simulink model "VSDk_PMSM_6"  (R2024a)
settings: Solver=VariableStepAuto  StartTime=0.0  StopTime=10.0  RelTol=1e-3
values from neighbouring files (symbols this model uses):
  faif = 0.1351    [init.m]
  Iq_limit = Tn/(1.5*p*faif)*1    (= 90.6192943499)    [init.m]
  Jm = 0.36    [init.m]
  Ki_id_vsd = Rs * wc    (= 61.7197292724)    [init.m]
  Ki_iq_vsd = Rs * wc    (= 61.7197292724)    [init.m]
  Ki_x = Rs * wc_xy    (= 61.7197292724)    [init.m]
  Ki_y = Rs * wc_xy    (= 61.7197292724)    [init.m]
  Kis_vsd = (ws^2 * Jm) / KT    (= 438.324399752)    [init.m]
  Kp_id_vsd = Ld_eff * wc    (= 0.485061905714)    [init.m]
  Kp_iq_vsd = Lq_eff * wc    (= 0.485061905714)    [init.m]
  Kp_x = Lx * wc_xy    (= 0.020106192983)    [init.m]
  Kp_y = Ly * wc_xy    (= 0.020106192983)    [init.m]
  Kps_vsd = (2 * zeta * ws * Jm) / KT    (= 19.7285507573)    [init.m]
  LD = Ld+Ldd    (= 7.72e-05)    [init.m]
  Ld = 40.2e-6    (= 4.02e-05)    [init.m]
  Ldd = 37e-6    (= 3.7e-05)    [init.m]
  Ldz = Ld-Ldd    (= 3.2e-06)    [init.m]
  LQ = Lq+Lqq    (= 7.72e-05)    [init.m]
  Lq = 40.2e-6    (= 4.02e-05)    [init.m]
  Lqq = 37e-6    (= 3.7e-05)    [init.m]
  n = 2000    [init.m]
  p = 4    [init.m]
  Rs = 9.823e-3    (= 0.009823)    [init.m]
  Tn = 734.56/10    (= 73.456)    [init.m]
  Ts = 1/(16e3)    (= 6.25e-05)    [init.m]
  Ts_FEA = 1e-7    (= 1e-07)    [init.m]
  VDC = 1200    [init.m]
  wc_xy = 2 * pi * fc_xy    (= 6283.18530718)    [init.m]
libraries: spsIGBTDiodeLib x24, spsVoltageMeasurementLib x16, spsSeriesRLCBranchLib x12, spsDiodeLib x12, spsOnDelayLib x12, slpidlib x11, simulink x7, spsControlledCurrentSourceLib x6, spsDCVoltageSourceLib x1, spsdq0toAlphaBetaZeroLib x1, spspowerguiLib x1
(part 3 of 3)

== matlab function VSDk_PMSM_6/Subsystem2/NTSV_9_nearest2 ==
  data: Alpha input; Beta input; Ta1 output; Ta2 output; Tb1 output; Tb2 output; Tc1 output; Tc2 output; r input; VecSector1 output
function [Ta1,Ta2,Tb1,Tb2,Tc1,Tc2,VecSector1]  = fcn(Alpha,Beta,r)
temp1=Beta;
temp2=0.8660254*Alpha+Beta*0.5;
temp3=temp2-temp1;
%0.8660254*Alpha-0.5beta
%temp1+temp2 0.8660254*Alpha+1.5beta
%temp3+temp2 2*0.8660254*Alpha
%temp1-temp3 -0.8660254*Alpha+1.5beta
VecSector1=3;
VecSector2=1;
VecSector3=0;


if temp2>0
    VecSector1=VecSector1-1;
end
if temp3>0
    VecSector1=VecSector1-1;
end
if temp1<0
    VecSector1=7-VecSector1;
end 


switch VecSector1
    case {1,4}  
       if(abs(temp2)>0.5)
           VecSector2=VecSector2+1;
           if(abs(temp3)<0.5)
               VecSector2=VecSector2+1;
               if(abs(temp1)>0.5)
                   VecSector2=VecSector2+1;
               end
           end
       end
       if(temp1<temp3)
           VecSector3=1;
       else
           VecSector3=2;
       end
    case {2,5}
       if(abs(temp1)>0.5)
           VecSector2=VecSector2+1;
           if(abs(temp2)<0.5)
               VecSector2=VecSector2+1;
               if(abs(temp3)>0.5)
                   VecSector2=VecSector2+1;
               end
           end
       end
       if(temp2+temp3>0)
          VecSector3=1;
       else
           VecSector3=2;
       end 
    case {3,6}
       if(abs(temp3)>0.5)
           VecSector2=VecSector2+1;
           if(abs(temp1)<0.5)
               VecSector2=VecSector2+1;
               if(abs(temp2)>0.5)
                   VecSector2=VecSector2+1;
               end
           end
       end
       if(temp1+temp2>0)
          VecSector3=1;
       else
           VecSector3=2;
       end 
    otherwise
        VecSector1=0;
        VecSector2=0;
end


switch VecSector1
    case 1
        Ta1=temp2;
        Ta2=1;
        Tc1=0;
        Tc2=1-temp2;
        switch VecSector2
            case 1
                Tb1=temp1;
                Tb2=1-temp3;
            case 2
                Tb1=0;
                Tb2=1+temp1-temp3;
            case 3
                Tb1=0.5-temp3;
                Tb2=0.5+temp1;
            case 4
                Tb1=temp1-temp3;
                Tb2=1;
            otherwise
                Tb1=0;
                Tb2=1;
        end
        if(VecSector3==1)
            Ta1=Ta1+Tc2*r;
            Tb2=Tb2+Tc2*r;
            Tc2=Tc2+Tc2*r;
        else
            Ta1=Ta1+Tc2*r;
            Tb1=Tb1+Tc2*r;
            Tc2=Tc2+Tc2*r;
        end
%--------------------------------------------------%
    case 2
        Tb1=temp1;
        Tb2=1;
        Tc1=0;
        Tc2=1-temp1;
        switch VecSector2
            case 1
                Ta1=temp2;
                Ta2=1+temp3;
            case 2
                Ta1=temp2+temp3;
                Ta2=1;
            case 3
                Ta1=0.5+temp3;
                Ta2=0.5+temp2;
            case 4
                Ta1=0;
                Ta2=1+temp2+temp3;
            otherwise
                Ta1=0;
                Ta2=1;
        end
        if(VecSector3==1)
            Ta1=Ta1+Tc2*r;
            Tb1=Tb1+Tc2*r;
            Tc2=Tc2+Tc2*r;
        else
            Ta2=Ta2+Tc2*r;
            Tb1=Tb1+Tc2*r;
            Tc2=Tc2+Tc2*r;
        end
%--------------------------------------------------%
    case 3
        Ta1=0;
        Ta2=1+temp3;
        Tb1=-temp3;
        Tb2=1;
        switch VecSector2
            case 1
                Tc1=-temp2;
                Tc2=1-temp1;
            case 2
                Tc1=0;
                Tc2=1-temp1-temp2;
            case 3
                Tc1=0.5-temp1;
                Tc2=0.5-temp2;
            case 4
                Tc1=-temp1-temp2;
                Tc2=1;
            otherwise
                Tc1=0;
                Tc2=1;
        end
        if(VecSector3==1)
            Tb1=Tb1+Ta2*r;
            Tc2=Tc2+Ta2*r;
            Ta2=Ta2+Ta2*r;
        else
            Tb1=Tb1+Ta2*r;
            Tc1=Tc1+Ta2*r;
            Ta2=Ta2+Ta2*r;
        end
%--------------------------------------------------%
    case 4
        Ta1=0;
        Ta2=1+temp2;
        Tc1=-temp2;
        Tc2=1;
        switch VecSector2
            case 1
                Tb1=-temp3;
                Tb2=1+temp1;
            case 2
                Tb1=temp1-temp3;
                Tb2=1;
            case 3
                Tb1=0.5+temp1;
                Tb2=0.5-temp3;
            case 4
                Tb1=0;
                Tb2=1+temp1-temp3;
            otherwise
                Tb1=0;
                Tb2=1;
        end
        if(VecSector3==1)
            Tb1=Tb1+Ta2*r;
            Tc1=Tc1+Ta2*r;
            Ta2=Ta2+Ta2*r;
        else
            Tb2=Tb2+Ta2*r;
            Tc1=Tc1+Ta2*r;
            Ta2=Ta2+Ta2*r;
        end
%--------------------------------------------------%
    case 5
        Tb1=0;
        Tb2=1+temp1;
        Tc1=-temp1;
        Tc2=1;
        switch VecSector2
            case 1
                Ta1=temp3;
                Ta2=1+temp2;
            case 2
                Ta1=0;
                Ta2=1+temp2+temp3;
            case 3
                Ta1=0.5+temp2;
                Ta2=0.5+temp3;
            case 4
                Ta1=temp2+temp3;
                Ta2=1;
            otherwise
                Ta1=0;
                Ta2=1;
        end
        if(VecSector3==1)
            Ta2=Ta2+Tb2*r;
            Tc1=Tc1+Tb2*r;
            Tb2=Tb2+Tb2*r;
        else
            Ta1=Ta1+Tb2*r;
            Tc1=Tc1+Tb2*r;
            Tb2=Tb2+Tb2*r;
        end
%--------------------------------------------------%
    case 6
        Ta1=temp3;
        Ta2=1;
        Tb1=0;
        Tb2=1-temp3;
        switch VecSector2
            case 1
                Tc1=-temp1;
                Tc2=1-temp2;
            case 2
                Tc1=-temp1-temp2;
                Tc2=1;
            case 3
                Tc1=0.5-temp2;
                Tc2=0.5-temp1;
            case 4
                Tc1=0;
                Tc2=1-temp1-temp2;
            otherwise
                Tc1=0;
                Tc2=1;
        end
        if(VecSector3==1)
            Ta1=Ta1+Tb2*r;
            Tc1=Tc1+Tb2*r;
            Tb2=Tb2+Tb2*r;
        else
            Ta1=Ta1+Tb2*r;
            Tc2=Tc2+Tb2*r;
            Tb2=Tb2+Tb2*r;
        end
%--------------------------------------------------%
    otherwise
        Ta1=0;
        Ta2=1;
        Tb1=0;
        Tb2=1;
        Tc1=0;
        Tc2=1;
end

== matlab function VSDk_PMSM_6/current regulator_Winding3/current regulator1/MATLAB Function ==
  data: uq_in input; uq output; ud_in input; ud output; VDC input
function [uq,ud] = overmodulation(uq_in,ud_in,VDC)

VDC_phase=VDC*0.5773502;
Uout=sqrt(ud_in*ud_in+uq_in*uq_in);

if(Uout>=VDC_phase*0.95)
    ud=ud_in/Uout;
    uq=uq_in/Uout;
else
    ud=ud_in/VDC_phase;
    uq=uq_in/VDC_phase;
end
end

== matlab function VSDk_PMSM_6/current regulator_Winding3/current regulator3/MATLAB Function ==
  data: uq_in input; uq output; ud_in input; ud output; VDC input
function [uq,ud] = overmodulation(uq_in,ud_in,VDC)

VDC_phase=VDC*0.5773502;
Uout=sqrt(ud_in*ud_in+uq_in*uq_in);

if(Uout>=VDC_phase*0.99)
    ud=ud_in/Uout;
    uq=uq_in/Uout;
else
    ud=ud_in/VDC_phase;
    uq=uq_in/VDC_phase;
end
end

== matlab function VSDk_PMSM_6/current regulator_Winding3/current regulator3/MATLAB Function1 ==
  data: i_meas input; d_est output; u_prev input; R input; L input; Ts input; wo input; z1_old input; z1_new output; z2_old input; z2_new output
function [d_est, z1_new, z2_new] = eso_observer(i_meas, u_prev, R, L, Ts, wo, z1_old, z2_old)
% ESO_OBSERVER 线性扩张状态观测器 (LESO)
%
% 输入参数:
%   i_meas  : 当前采样的电流值 (Amps)
%   u_prev  : 上一时刻施加的电压值 (Volts) -> 导致产生当前电流的电压
%   z_prev  : 上一时刻的观测器状态向量 [2x1] -> [估计电流; 估计扰动]
%   param   : 参数结构体，包含 R, L, Ts, omega_o
%
% 输出参数:
%   d_est   : 估计出的扰动值 (Volts)
%   z_next  : 更新后的观测器状态向量 [2x1] -> 供下一时刻迭代使用

    % 2. 计算观测器增益 (极点配置法)
    % 特征方程: (s + wo)^2 = s^2 + 2*wo*s + wo^2
    % 对应误差动态方程，推导出的增益如下：
    beta1 = 2 * wo - (R / L);  % 电流状态增益
    beta2 = L * wo^2;          % 扰动状态增益

    % 4. 计算估计误差
    % e = 实际测量值 - 估计值
    e = i_meas - z1_old;

    % 5. 更新状态 (使用前向欧拉法离散化)
    % 状态方程: 
    % dz1/dt = (u - R*z1 + z2)/L + beta1*e
    % dz2/dt = beta2 * e
    
    % 计算微分量
    dz1 = (u_prev - R * z1_old + z2_old) / L + beta1 * e;
    dz2 = beta2 * e;

    % 积分更新
    z1_new = z1_old + Ts * dz1;
    z2_new = z2_old + Ts * dz2;
    
    % 输出当前的扰动估计值 (z2)
    % 注意：这里输出 z2_new 代表最实时的估计
    d_est = z2_new; 
end

== matlab function VSDk_PMSM_6/current regulator_Winding3/current regulator3/MATLAB Function2 ==
  data: i_meas input; d_est output; u_prev input; R input; L input; Ts input; wo input; z1_old input; z1_new output; z2_old input; z2_new output
function [d_est, z1_new, z2_new] = eso_observer(i_meas, u_prev, R, L, Ts, wo, z1_old, z2_old)
% ESO_OBSERVER 线性扩张状态观测器 (LESO)
%
% 输入参数:
%   i_meas  : 当前采样的电流值 (Amps)
%   u_prev  : 上一时刻施加的电压值 (Volts) -> 导致产生当前电流的电压
%   z_prev  : 上一时刻的观测器状态向量 [2x1] -> [估计电流; 估计扰动]
%   param   : 参数结构体，包含 R, L, Ts, omega_o
%
% 输出参数:
%   d_est   : 估计出的扰动值 (Volts)
%   z_next  : 更新后的观测器状态向量 [2x1] -> 供下一时刻迭代使用

    % 2. 计算观测器增益 (极点配置法)
    % 特征方程: (s + wo)^2 = s^2 + 2*wo*s + wo^2
    % 对应误差动态方程，推导出的增益如下：
    beta1 = 2 * wo - (R / L);  % 电流状态增益
    beta2 = L * wo^2;          % 扰动状态增益

    % 4. 计算估计误差
    % e = 实际测量值 - 估计值
    e = i_meas - z1_old;

    % 5. 更新状态 (使用前向欧拉法离散化)
    % 状态方程: 
    % dz1/dt = (u - R*z1 + z2)/L + beta1*e
    % dz2/dt = beta2 * e
    
    % 计算微分量
    dz1 = (u_prev - R * z1_old + z2_old) / L + beta1 * e;
    dz2 = beta2 * e;

    % 积分更新
    z1_new = z1_old + Ts * dz1;
    z2_new = z2_old + Ts * dz2;
    
    % 输出当前的扰动估计值 (z2)
    % 注意：这里输出 z2_new 代表最实时的估计
    d_est = z2_new; 
end
